simulink model "Thermal_Model_v5"  (R2026a)
settings: Solver=ode23t  StopTime=900
model workspace (MAT data in the model file):
  Area_coolant_bottom_port_in_m2 = 7.85398163397e-05
  Area_coolant_top_port_in_m2 = 7.85398163397e-05
  CurrentProfile = [0  80; 300  80; 300  0; 600  0; 600  -80; 900  -80]
  SOC0 = 0.4
  T_ambient_K = 298.15
  T_coolant_bottom_in_K = 298.15
  T_coolant_top_in_K = 298.15
  mdot_coolant_bottom = 0.02
  mdot_coolant_top = 0.02
libraries: fl_lib x24, nesl_utility x21, ThermalPackComponents_lib x6, batt_lib x6, SimscapeFluids_lib x6, Cylindrical_Cell_Module_v2_5_lib x1
settings Model: LastModifiedBy=Talha

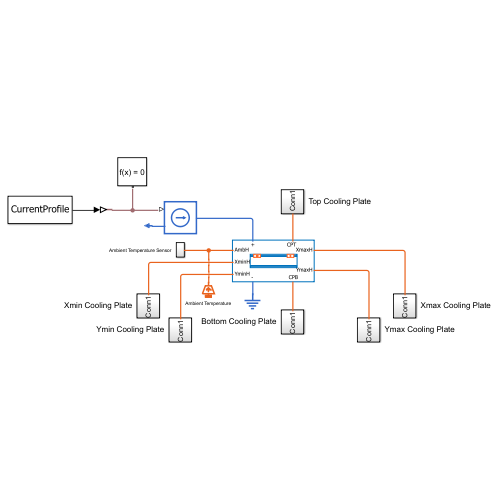
[thumbnail: Simulink's stored preview of the top-level diagram]
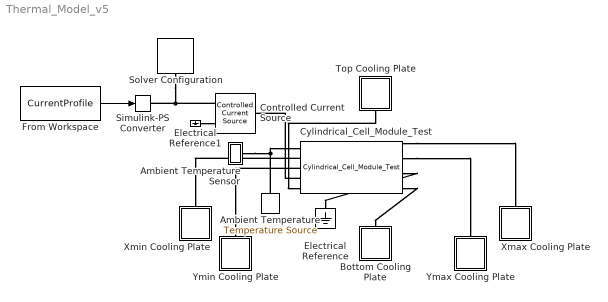
== system Thermal_Model_v5 ==
  Ambient Temperature : fl_lib/Thermal/Thermal Sources/Temperature Source  temperature=T_ambient_K K
  Ambient Temperature Sensor : Subsystem
  Bottom Cooling Plate : Subsystem
  Controlled Current Source : fl_lib/Electrical/Electrical Sources/Controlled Current Source
  Cylindrical_Cell_Module_Test : Cylindrical_Cell_Module_v2_5_lib/Cylindrical_Cell_Module_Test  BatteryCapacityCell=5 A*hr  BatteryCapacityCellPercentDeviation=zeros([12, 1])  ExtrapolationMethodCell=simscape.enum.extrapolation.nearest  SOCBreakpointsCell=[0, .1, .25, .5, .75, .9, 1]  SOCBreakpointsCellPercentDeviation=zeros([12, 1])  TemperatureBreakpointsCell=[278, 293, 313] K  TemperatureBreakpointsCellPercentDeviation=zeros([12, 1])  OpenCircuitVoltageThermalCell=[3.49, 3.5, 3.51; 3.55, 3.57, 3.56; 3.62, 3.63, 3.64; 3.71, 3.71, 3.72; 3.91, 3.93, 3.94; 4.07, 4.08, 4.08; 4.19, 4.19, 4.19] V  OpenCircuitVoltageThermalCellPercentDeviation=zeros([12, 1])  VoltageRangeCell=[0, inf] V  VoltageRangeCellPercentDeviation=zeros([12, 1])  ResistanceSOCBreakpointsCell=[0, .1, .25, .5, .75, .9, 1]  ResistanceSOCBreakpointsCellPercentDeviation=zeros([12, 1])  ResistanceTemperatureBreakpointsCell=[278, 293, 313] K  ResistanceTemperatureBreakpointsCellPercentDeviation=zeros([12, 1])  R0ThermalCell=[.0117, .0085, .009; .011, .0085, .009; .0114, .0087, .0092; .0107, .0082, .0088; .0107, .0083, .0091; .0113, .0085, .0089; .0116, .0085, .0089] Ohm  R0ThermalCellPercentDeviation=zeros([12, 1])  BatteryThermalMassCell=100 J/K  BatteryThermalMassCellPercentDeviation=zeros([12, 1])  NumThermalModelsCell=6  NumThermalModelsCellPercentDeviation=zeros([12, 1])  ThermalConductivityZCell=15 W/(K*m)  ThermalConductivityZCellPercentDeviation=zeros([12, 1])  CrossSectionalAreaXYCell=3.142e-4 m^2  CrossSectionalAreaXYCellPercentDeviation=zeros([12, 1])  HeightCell=0.07 m  HeightCellPercentDeviation=zeros([12, 1])  CoolantResistance=1.2 K/W  AmbientResistance=25 K/W  XminThermalResistance=25 K/W  XmaxThermalResistance=25 K/W  YminThermalResistance=25 K/W  YmaxThermalResistance=25 K/W  InterCellThermalResistance=1 K/W  InterParallelAssemblyThermalResistance=1 K/W  socCell_specify=on  socCell_priority=High  socCell=repmat(0.4, 12, 1)  socCell_nominal_specify=off  socCell_nominal_value=1  socCell_nominal_unit=1  batteryVoltage_specify=off  batteryVoltage_priority=None  batteryVoltage=repmat(0, 12, 1) V  batteryVoltage_nominal_specify=off  batteryVoltage_nominal_value=1  batteryVoltage_nominal_unit=V  batteryCurrent_specify=off  batteryCurrent_priority=None  batteryCurrent=repmat(0, 12, 1) A  batteryCurrent_nominal_specify=off  batteryCurrent_nominal_value=1  batteryCurrent_nominal_unit=A  numCycles_specify=off  numCycles_priority=High  numCycles=repmat(0, 12, 1)  numCycles_nominal_specify=off  numCycles_nominal_value=1  numCycles_nominal_unit=1  batteryTemperature_specify=on  batteryTemperature_priority=High  batteryTemperature=repmat(298.15, 12, 1) K  batteryTemperature_nominal_specify=off  batteryTemperature_nominal_value=1  batteryTemperature_nominal_unit=K  vParallelAssembly_specify=off  vParallelAssembly_priority=None  vParallelAssembly=repmat(0, 3, 1) V  vParallelAssembly_nominal_specify=off  vParallelAssembly_nominal_value=1  vParallelAssembly_nominal_unit=V  socParallelAssembly_specify=off  socParallelAssembly_priority=None  socParallelAssembly=repmat(1, 3, 1)  socParallelAssembly_nominal_specify=off  socParallelAssembly_nominal_value=1  socParallelAssembly_nominal_unit=1
  Electrical Reference : fl_lib/Electrical/Electrical Elements/Electrical Reference
  Electrical Reference1 : fl_lib/Electrical/Electrical Elements/Electrical Reference
  From Workspace : FromWorkspace  VariableName=CurrentProfile  Interpolate=off  OutputAfterFinalValue=Holding final value
  Simulink-PS Converter : nesl_utility/Simulink-PS Converter  PhysicalDomain=network_engine_domain  SubClassName=ps_input  LeftPortType=input  RightPortType=output  PseudoPeriodic=off  Frequencies=[]  NoiseDistribution=none  NoiseParameters=[]  Unit=1  AffineConversion=off  FilteringAndDerivatives=provide  SimscapeFilterOrder=1  InputFilterTimeConstant=0.001  UdotUserProvided=0
  Solver Configuration : nesl_utility/Solver Configuration  PhysicalDomain=network_engine_domain  SubClassName=solver  LeftPortType=input  RightPortType=generic  Tones=[]  Harmonics=[]  SimulateNoise=off  Profile=off  UseLocalSampling=off  EnableSwitchedLinearOptims=on  FrequencyDomain=off  UseCCode=off  RelTol=0.001  AbsTol=0.001  MinStep=1e-09  ToWorkspace=off  RevertToSquareIcSolve=off  NumHomotopyIterations=100  PhasorMode=off  PhasorModeNumHarmonics=1  ConsistencySolver=NEWTON_XTOL_AFTER_FTOL  CanonicalOrdering=CANONICAL  OptimizeIntermediates=OPTIMIZED  IndexReductionMethod=DerivativeReplacement  DoDC=off  ResidualTolerance=1e-09  ConsistencyTolSource=GLOBAL  ConsistencyAbsTol=0.001  ConsistencyRelTol=0.001  ConsistencyTolFactor=0.001  UseLocalSolver=off  LocalSolverChoice=NE_BACKWARD_EULER_ADVANCER  ResolveIndetEquations=on  FunctionEvalNumThread=1  LocalSolverSampleTime=0.001  DoFixedCost=off  MaxNonlinIter=3  MaxModeIter=2  ComputeImpulses=off  ImpulseIterations=2  LinearAlgebra=auto  LinearAlgebraNumThread=0  EquationFormulation=NE_TIME_EF  DelaysMemoryBudget=1024  AutomaticFiltering=on  FilteringTimeConstant=0.001  PartitionStorageMethod=AS_NEEDED  PartitionMemoryBudget=1024  PartitionMethod=ROBUST  MultibodyUseLocalSolver=off  MultibodyLocalSolverChoice=ODE1  MultibodyLocalSolverSampleTime=0.001
  Top Cooling Plate : Subsystem
  Xmax Cooling Plate : Subsystem
  Xmin Cooling Plate : Subsystem
  Ymax Cooling Plate : Subsystem
  Ymin Cooling Plate : Subsystem
  wires:
  From Workspace/1 -> Simulink-PS Converter/1
  connections:
  Controlled Current Source/RConn1 -- Solver Configuration/RConn1 -- Simulink-PS Converter/RConn1
  Cylindrical_Cell_Module_Test/RConn3 -- Electrical Reference/LConn1
  Cylindrical_Cell_Module_Test/LConn4 -- Controlled Current Source/LConn1
  Electrical Reference1/LConn1 -- Controlled Current Source/RConn2
  Ambient Temperature Sensor/LConn1 -- Ambient Temperature/LConn1 -- Cylindrical_Cell_Module_Test/LConn1
  Top Cooling Plate/LConn1 -- Cylindrical_Cell_Module_Test/LConn5
  Cylindrical_Cell_Module_Test/RConn4 -- Bottom Cooling Plate/LConn1
  Cylindrical_Cell_Module_Test/LConn2 -- Xmin Cooling Plate/LConn1
  Cylindrical_Cell_Module_Test/LConn3 -- Ymin Cooling Plate/LConn1
  Cylindrical_Cell_Module_Test/RConn1 -- Xmax Cooling Plate/LConn1
  Cylindrical_Cell_Module_Test/RConn2 -- Ymax Cooling Plate/LConn1

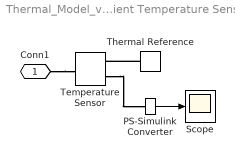
== system Thermal_Model_v5/Ambient Temperature Sensor ==
  PS-Simulink Converter : nesl_utility/PS-Simulink Converter  PhysicalDomain=network_engine_domain  SubClassName=ps_output  LeftPortType=input  RightPortType=output  PseudoPeriodic=off  Frequencies=[]  VectorFormat=inherit  Unit=inherit  AffineConversion=off
  Scope : Scope
      settings: ActiveDisplayYMinimum=-1  ActiveDisplayYMaximum=1
  Temperature Sensor : fl_lib/Thermal/Thermal Sensors/Temperature Sensor  temperature_measure=foundation.enum.MeasurementReference.difference
  Thermal Reference : fl_lib/Thermal/Thermal Elements/Thermal Reference
  Conn1 : PMIOPort  Side=Left
  wires:
  PS-Simulink Converter/1 -> Scope/1
  connections:
  Thermal Reference/LConn1 -- Temperature Sensor/RConn1
  Temperature Sensor/RConn2 -- PS-Simulink Converter/LConn1
  Conn1/RConn1 -- Temperature Sensor/LConn1

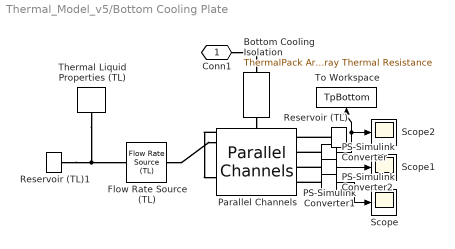
== system Thermal_Model_v5/Bottom Cooling Plate ==
  Bottom Cooling Isolation : ThermalPackComponents_lib/ThermalPack Array Thermal Resistance  N=12  R=1e-6 K/W
  Flow Rate Source (TL) : fl_lib/Thermal Liquid/Sources/Flow Rate Source (TL)  source_type=foundation.enum.constant_controlled.constant  flow_type=foundation.enum.mass_volumetric_flow.mass  mass_flow=mdot_coolant_bottom kg/s  volumetric_flow=0 m^3/s  power_spec=foundation.enum.power_spec.none  area=Area_coolant_bottom_port_in_m2 m^2
  PS-Simulink Converter : nesl_utility/PS-Simulink Converter  PhysicalDomain=network_engine_domain  SubClassName=ps_output  LeftPortType=input  RightPortType=output  PseudoPeriodic=off  Frequencies=[]  VectorFormat=inherit  Unit=inherit  AffineConversion=off
  PS-Simulink Converter1 : nesl_utility/PS-Simulink Converter  PhysicalDomain=network_engine_domain  SubClassName=ps_output  LeftPortType=input  RightPortType=output  PseudoPeriodic=off  Frequencies=[]  VectorFormat=inherit  Unit=inherit  AffineConversion=off
  PS-Simulink Converter2 : nesl_utility/PS-Simulink Converter  PhysicalDomain=network_engine_domain  SubClassName=ps_output  LeftPortType=input  RightPortType=output  PseudoPeriodic=off  Frequencies=[]  VectorFormat=inherit  Unit=inherit  AffineConversion=off
  Parallel Channels : batt_lib/Thermal/Parallel Channels  plateConnectivity=simscape.battery.enum.thermal.coolingPlateConnectivity.singleSided  numBattThermalNodes1=12  dimensionThermalNodes1=[0.0200 0.0200; 0.0200 0.0200; 0.0200 0.0200; 0.0200 0.0200; 0.0200 0.0200; 0.0200 0.0200; 0.0200 0.0200; 0.0200 0.0200; 0.0200 0.0200; 0.0200 0.0200; 0.0200 0.0200; 0.0200 0.0200]  locationThermalNodes1=[0.0100 0.0100; 0.0100 0.0310; 0.0100 0.0520; 0.0100 0.0730; 0.0310 0.0100; 0.0310 0.0310; 0.0310 0.0520; 0.0310 0.0730; 0.0520 0.0100; 0.0520 0.0310; 0.0520 0.0520; 0.0520 0.0730]  numBattThermalNodes2=1  dimensionThermalNodes2=ones(1, 2)  locationThermalNodes2=ones(1, 2)  plateDimX=3  plateDimY=4  plateTh=2e-3 m  plateThCond=205 W/(K*m)  plateDen=2700 kg/m^3  plateCp=900 J/(K*kg)  plateTemp_ini=298.15 K  Re_lam=2000  Re_tur=4000  Nu_lam=3.66  length_add=1e-3 m  shape_factor=64  nChannels=4  selectChannelOrientation=simscape.battery.enum.thermal.coolingChannelsDirection.alongX  channelDia=0.004 m  distributorDia=0.006 m  roughnessPipe=1.5e-05 m
  Reservoir (TL) : fl_lib/Thermal Liquid/Elements/Reservoir (TL)  pressure_input=false  pressure_spec=foundation.enum.pressure_spec.atmospheric  reservoir_pressure=101325 Pa  temperature_input=false  reservoir_temperature=298.15 K  area=Area_coolant_bottom_port_in_m2 m^2  input_error_spec=foundation.enum.input_range_error.warn
  Reservoir (TL)1 : fl_lib/Thermal Liquid/Elements/Reservoir (TL)  pressure_input=false  pressure_spec=foundation.enum.pressure_spec.atmospheric  reservoir_pressure=101325 Pa  temperature_input=false  reservoir_temperature=T_coolant_bottom_in_K K  area=Area_coolant_bottom_port_in_m2 m^2  input_error_spec=foundation.enum.input_range_error.warn
  Scope : Scope
      settings: ActiveDisplayYMinimum=-5455.2115602984395  ActiveDisplayYMaximum=-5434.2762079587283
  Scope1 : Scope
      settings: ActiveDisplayYMinimum=-1  ActiveDisplayYMaximum=1  DataLoggingVariableName=ScopeData2
  Scope2 : Scope
      settings: ActiveDisplayYMinimum=300.00863941911916  ActiveDisplayYMaximum=300.14142336544342  DataLoggingVariableName=ScopeData3
  Thermal Liquid Properties (TL) : SimscapeFluids_lib/Thermal Liquid/Utilities/Thermal Liquid Properties (TL)  fluid_list=fluids.thermal_liquid.utilities.enum.thermal_liquid_fluid_list.ethylene_glycol  concentration_param_EG=fluids.thermal_liquid.utilities.enum.thermal_liquid_concentration.volume_fraction  concentration_param_PG=fluids.thermal_liquid.utilities.enum.thermal_liquid_concentration.volume_fraction  c_mass_SW=3.5e-3  c_mass_EG=0.1  c_mass_PG=0.1  c_mass_GL=0.1  c_vol_EG=0.5  c_vol_PG=0.1  beta_const_EG=2.1791 GPa  beta_const_PG=2.1791 GPa  beta_const_GL=2.1791 GPa  p_min_EG=0.01 MPa  p_min_PG=0.01 MPa  p_min_GL=0.01 MPa  p_max_EG=50 MPa  p_max_PG=50 MPa  p_max_GL=50 MPa  T_atm=298.15 K  p_atm=0.101325 MPa  properties_range_check=simscape.enum.assert.action.error  air_fraction=0.005  R_air=0.287 kJ/(K*kg)  air_dissolution_model=false  p_crit=3 MPa
  To Workspace : ToWorkspace  VariableName=TpBottom  SaveFormat=Timeseries  SampleTime=-1
  Conn1 : PMIOPort  Side=Left
  wires:
  PS-Simulink Converter/1 -> Scope2/1, To Workspace/1
  PS-Simulink Converter1/1 -> Scope1/1
  PS-Simulink Converter2/1 -> Scope/1
  connections:
  PS-Simulink Converter2/LConn1 -- Parallel Channels/RConn4
  Reservoir (TL)1/LConn1 -- Thermal Liquid Properties (TL)/RConn1 -- Flow Rate Source (TL)/LConn1
  PS-Simulink Converter1/LConn1 -- Parallel Channels/RConn3
  PS-Simulink Converter/LConn1 -- Parallel Channels/RConn2
  Reservoir (TL)/LConn1 -- Parallel Channels/RConn1
  Bottom Cooling Isolation/RConn1 -- Parallel Channels/LConn2
  Flow Rate Source (TL)/RConn1 -- Parallel Channels/LConn1
  Conn1/RConn1 -- Bottom Cooling Isolation/LConn1

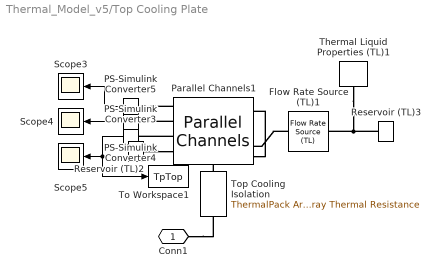
== system Thermal_Model_v5/Top Cooling Plate ==
  Flow Rate Source (TL)1 : fl_lib/Thermal Liquid/Sources/Flow Rate Source (TL)  source_type=foundation.enum.constant_controlled.constant  flow_type=foundation.enum.mass_volumetric_flow.mass  mass_flow=mdot_coolant_top kg/s  volumetric_flow=0 m^3/s  power_spec=foundation.enum.power_spec.none  area=Area_coolant_top_port_in_m2 m^2
  PS-Simulink Converter3 : nesl_utility/PS-Simulink Converter  PhysicalDomain=network_engine_domain  SubClassName=ps_output  LeftPortType=input  RightPortType=output  PseudoPeriodic=off  Frequencies=[]  VectorFormat=inherit  Unit=inherit  AffineConversion=off
  PS-Simulink Converter4 : nesl_utility/PS-Simulink Converter  PhysicalDomain=network_engine_domain  SubClassName=ps_output  LeftPortType=input  RightPortType=output  PseudoPeriodic=off  Frequencies=[]  VectorFormat=inherit  Unit=inherit  AffineConversion=off
  PS-Simulink Converter5 : nesl_utility/PS-Simulink Converter  PhysicalDomain=network_engine_domain  SubClassName=ps_output  LeftPortType=input  RightPortType=output  PseudoPeriodic=off  Frequencies=[]  VectorFormat=inherit  Unit=inherit  AffineConversion=off
  Parallel Channels1 : batt_lib/Thermal/Parallel Channels  plateConnectivity=simscape.battery.enum.thermal.coolingPlateConnectivity.singleSided  numBattThermalNodes1=12  dimensionThermalNodes1=[0.0200 0.0200; 0.0200 0.0200; 0.0200 0.0200; 0.0200 0.0200; 0.0200 0.0200; 0.0200 0.0200; 0.0200 0.0200; 0.0200 0.0200; 0.0200 0.0200; 0.0200 0.0200; 0.0200 0.0200; 0.0200 0.0200]  locationThermalNodes1=[0.0100 0.0100; 0.0100 0.0310; 0.0100 0.0520; 0.0100 0.0730; 0.0310 0.0100; 0.0310 0.0310; 0.0310 0.0520; 0.0310 0.0730; 0.0520 0.0100; 0.0520 0.0310; 0.0520 0.0520; 0.0520 0.0730]  numBattThermalNodes2=1  dimensionThermalNodes2=ones(1, 2)  locationThermalNodes2=ones(1, 2)  plateDimX=3  plateDimY=4  plateTh=2e-3 m  plateThCond=205 W/(K*m)  plateDen=2700 kg/m^3  plateCp=900 J/(K*kg)  plateTemp_ini=298.15 K  Re_lam=2000  Re_tur=4000  Nu_lam=3.66  length_add=1e-3 m  shape_factor=64  nChannels=4  selectChannelOrientation=simscape.battery.enum.thermal.coolingChannelsDirection.alongX  channelDia=0.004 m  distributorDia=0.006 m  roughnessPipe=1.5e-05 m
  Reservoir (TL)2 : fl_lib/Thermal Liquid/Elements/Reservoir (TL)  pressure_input=false  pressure_spec=foundation.enum.pressure_spec.atmospheric  reservoir_pressure=101325 Pa  temperature_input=false  reservoir_temperature=298.15 K  area=Area_coolant_top_port_in_m2 m^2  input_error_spec=foundation.enum.input_range_error.warn
  Reservoir (TL)3 : fl_lib/Thermal Liquid/Elements/Reservoir (TL)  pressure_input=false  pressure_spec=foundation.enum.pressure_spec.atmospheric  reservoir_pressure=101325 Pa  temperature_input=false  reservoir_temperature=T_coolant_top_in_K K  area=Area_coolant_top_port_in_m2 m^2  input_error_spec=foundation.enum.input_range_error.warn
  Scope3 : Scope
      settings: ActiveDisplayYMinimum=-5455.2115602984395  ActiveDisplayYMaximum=-5434.2762079587283  DataLoggingVariableName=ScopeData4
  Scope4 : Scope
      settings: ActiveDisplayYMinimum=-1  ActiveDisplayYMaximum=1  DataLoggingVariableName=ScopeData5
  Scope5 : Scope
      settings: ActiveDisplayYMinimum=300.00863941911916  ActiveDisplayYMaximum=300.14142336544342  DataLoggingVariableName=ScopeData6
  Thermal Liquid Properties (TL)1 : SimscapeFluids_lib/Thermal Liquid/Utilities/Thermal Liquid Properties (TL)  fluid_list=fluids.thermal_liquid.utilities.enum.thermal_liquid_fluid_list.ethylene_glycol  concentration_param_EG=fluids.thermal_liquid.utilities.enum.thermal_liquid_concentration.volume_fraction  concentration_param_PG=fluids.thermal_liquid.utilities.enum.thermal_liquid_concentration.volume_fraction  c_mass_SW=3.5e-3  c_mass_EG=0.1  c_mass_PG=0.1  c_mass_GL=0.1  c_vol_EG=0.5  c_vol_PG=0.1  beta_const_EG=2.1791 GPa  beta_const_PG=2.1791 GPa  beta_const_GL=2.1791 GPa  p_min_EG=0.01 MPa  p_min_PG=0.01 MPa  p_min_GL=0.01 MPa  p_max_EG=50 MPa  p_max_PG=50 MPa  p_max_GL=50 MPa  T_atm=298.15 K  p_atm=0.101325 MPa  properties_range_check=simscape.enum.assert.action.error  air_fraction=0.005  R_air=0.287 kJ/(K*kg)  air_dissolution_model=false  p_crit=3 MPa
  To Workspace1 : ToWorkspace  VariableName=TpTop  SaveFormat=Timeseries  SampleTime=-1
  Top Cooling Isolation : ThermalPackComponents_lib/ThermalPack Array Thermal Resistance  N=12  R=1e9 K/W
  Conn1 : PMIOPort  Side=Left
  wires:
  PS-Simulink Converter3/1 -> To Workspace1/1, Scope5/1
  PS-Simulink Converter5/1 -> Scope3/1
  PS-Simulink Converter4/1 -> Scope4/1
  connections:
  Reservoir (TL)2/LConn1 -- Parallel Channels1/RConn1
  Parallel Channels1/RConn4 -- PS-Simulink Converter5/LConn1
  Thermal Liquid Properties (TL)1/RConn1 -- Reservoir (TL)3/LConn1 -- Flow Rate Source (TL)1/LConn1
  Parallel Channels1/RConn3 -- PS-Simulink Converter4/LConn1
  Top Cooling Isolation/RConn1 -- Parallel Channels1/LConn2
  Parallel Channels1/RConn2 -- PS-Simulink Converter3/LConn1
  Flow Rate Source (TL)1/RConn1 -- Parallel Channels1/LConn1
  Conn1/RConn1 -- Top Cooling Isolation/LConn1

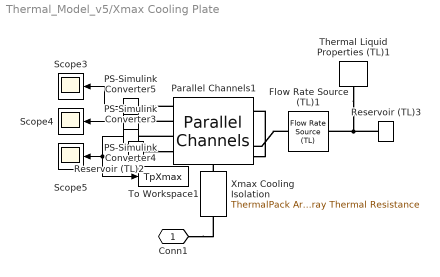
== system Thermal_Model_v5/Xmax Cooling Plate ==
  Flow Rate Source (TL)1 : fl_lib/Thermal Liquid/Sources/Flow Rate Source (TL)  source_type=foundation.enum.constant_controlled.constant  flow_type=foundation.enum.mass_volumetric_flow.mass  mass_flow=mdot_coolant_Xmax kg/s  volumetric_flow=0 m^3/s  power_spec=foundation.enum.power_spec.none  area=Area_coolant_Xmax_port_in_m2 m^2
  PS-Simulink Converter3 : nesl_utility/PS-Simulink Converter  PhysicalDomain=network_engine_domain  SubClassName=ps_output  LeftPortType=input  RightPortType=output  PseudoPeriodic=off  Frequencies=[]  VectorFormat=inherit  Unit=inherit  AffineConversion=off
  PS-Simulink Converter4 : nesl_utility/PS-Simulink Converter  PhysicalDomain=network_engine_domain  SubClassName=ps_output  LeftPortType=input  RightPortType=output  PseudoPeriodic=off  Frequencies=[]  VectorFormat=inherit  Unit=inherit  AffineConversion=off
  PS-Simulink Converter5 : nesl_utility/PS-Simulink Converter  PhysicalDomain=network_engine_domain  SubClassName=ps_output  LeftPortType=input  RightPortType=output  PseudoPeriodic=off  Frequencies=[]  VectorFormat=inherit  Unit=inherit  AffineConversion=off
  Parallel Channels1 : batt_lib/Thermal/Parallel Channels  plateConnectivity=simscape.battery.enum.thermal.coolingPlateConnectivity.singleSided  numBattThermalNodes1=4  dimensionThermalNodes1=|  locationThermalNodes1=|  numBattThermalNodes2=1  dimensionThermalNodes2=ones(1, 2)  locationThermalNodes2=ones(1, 2)  plateDimX=3  plateDimY=4  plateTh=2e-3 m  plateThCond=205 W/(K*m)  plateDen=2700 kg/m^3  plateCp=900 J/(K*kg)  plateTemp_ini=298.15 K  Re_lam=2000  Re_tur=4000  Nu_lam=3.66  length_add=1e-3 m  shape_factor=64  nChannels=4  selectChannelOrientation=simscape.battery.enum.thermal.coolingChannelsDirection.alongX  channelDia=0.004 m  distributorDia=0.006 m  roughnessPipe=1.5e-05 m
      dimensionThermalNodes1=|
      | [0.0700 0.0314; 0.0700 0.0314; 0.0700 0.0314;
      | 0.0700 0.0314]
      locationThermalNodes1=|
      | [0.0350 0.0100;
      | 0.0350 0.0310;
      | 0.0350 0.0520;
      | 0.0350 0.0730]
  Reservoir (TL)2 : fl_lib/Thermal Liquid/Elements/Reservoir (TL)  pressure_input=false  pressure_spec=foundation.enum.pressure_spec.atmospheric  reservoir_pressure=101325 Pa  temperature_input=false  reservoir_temperature=298.15 K  area=Area_coolant_Xmax_port_in_m2 m^2  input_error_spec=foundation.enum.input_range_error.warn
  Reservoir (TL)3 : fl_lib/Thermal Liquid/Elements/Reservoir (TL)  pressure_input=false  pressure_spec=foundation.enum.pressure_spec.atmospheric  reservoir_pressure=101325 Pa  temperature_input=false  reservoir_temperature=T_coolant_Xmax_in_K K  area=Area_coolant_Xmax_port_in_m2 m^2  input_error_spec=foundation.enum.input_range_error.warn
  Scope3 : Scope
      settings: ActiveDisplayYMinimum=-5455.2115602984395  ActiveDisplayYMaximum=-5434.2762079587283  DataLoggingVariableName=ScopeData4
  Scope4 : Scope
      settings: ActiveDisplayYMinimum=-1  ActiveDisplayYMaximum=1  DataLoggingVariableName=ScopeData5
  Scope5 : Scope
      settings: ActiveDisplayYMinimum=300.00863941911916  ActiveDisplayYMaximum=300.14142336544342  DataLoggingVariableName=ScopeData6
  Thermal Liquid Properties (TL)1 : SimscapeFluids_lib/Thermal Liquid/Utilities/Thermal Liquid Properties (TL)  fluid_list=fluids.thermal_liquid.utilities.enum.thermal_liquid_fluid_list.ethylene_glycol  concentration_param_EG=fluids.thermal_liquid.utilities.enum.thermal_liquid_concentration.volume_fraction  concentration_param_PG=fluids.thermal_liquid.utilities.enum.thermal_liquid_concentration.volume_fraction  c_mass_SW=3.5e-3  c_mass_EG=0.1  c_mass_PG=0.1  c_mass_GL=0.1  c_vol_EG=0.5  c_vol_PG=0.1  beta_const_EG=2.1791 GPa  beta_const_PG=2.1791 GPa  beta_const_GL=2.1791 GPa  p_min_EG=0.01 MPa  p_min_PG=0.01 MPa  p_min_GL=0.01 MPa  p_max_EG=50 MPa  p_max_PG=50 MPa  p_max_GL=50 MPa  T_atm=298.15 K  p_atm=0.101325 MPa  properties_range_check=simscape.enum.assert.action.error  air_fraction=0.005  R_air=0.287 kJ/(K*kg)  air_dissolution_model=false  p_crit=3 MPa
  To Workspace1 : ToWorkspace  VariableName=TpXmax  SaveFormat=Timeseries  SampleTime=-1
  Xmax Cooling Isolation : ThermalPackComponents_lib/ThermalPack Array Thermal Resistance  N=4  R=1e9 K/W
  Conn1 : PMIOPort  Side=Left
  wires:
  PS-Simulink Converter3/1 -> To Workspace1/1, Scope5/1
  PS-Simulink Converter5/1 -> Scope3/1
  PS-Simulink Converter4/1 -> Scope4/1
  connections:
  Reservoir (TL)2/LConn1 -- Parallel Channels1/RConn1
  Parallel Channels1/RConn4 -- PS-Simulink Converter5/LConn1
  Thermal Liquid Properties (TL)1/RConn1 -- Reservoir (TL)3/LConn1 -- Flow Rate Source (TL)1/LConn1
  Parallel Channels1/RConn3 -- PS-Simulink Converter4/LConn1
  Xmax Cooling Isolation/RConn1 -- Parallel Channels1/LConn2
  Parallel Channels1/RConn2 -- PS-Simulink Converter3/LConn1
  Flow Rate Source (TL)1/RConn1 -- Parallel Channels1/LConn1
  Conn1/RConn1 -- Xmax Cooling Isolation/LConn1

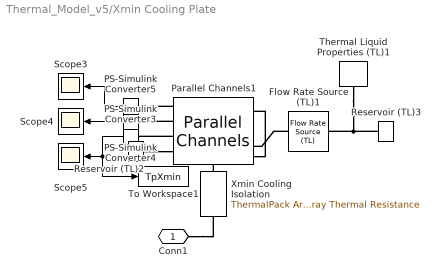
== system Thermal_Model_v5/Xmin Cooling Plate ==
  Flow Rate Source (TL)1 : fl_lib/Thermal Liquid/Sources/Flow Rate Source (TL)  source_type=foundation.enum.constant_controlled.constant  flow_type=foundation.enum.mass_volumetric_flow.mass  mass_flow=mdot_coolant_Xmin kg/s  volumetric_flow=0 m^3/s  power_spec=foundation.enum.power_spec.none  area=Area_coolant_Xmin_port_in_m2 m^2
  PS-Simulink Converter3 : nesl_utility/PS-Simulink Converter  PhysicalDomain=network_engine_domain  SubClassName=ps_output  LeftPortType=input  RightPortType=output  PseudoPeriodic=off  Frequencies=[]  VectorFormat=inherit  Unit=inherit  AffineConversion=off
  PS-Simulink Converter4 : nesl_utility/PS-Simulink Converter  PhysicalDomain=network_engine_domain  SubClassName=ps_output  LeftPortType=input  RightPortType=output  PseudoPeriodic=off  Frequencies=[]  VectorFormat=inherit  Unit=inherit  AffineConversion=off
  PS-Simulink Converter5 : nesl_utility/PS-Simulink Converter  PhysicalDomain=network_engine_domain  SubClassName=ps_output  LeftPortType=input  RightPortType=output  PseudoPeriodic=off  Frequencies=[]  VectorFormat=inherit  Unit=inherit  AffineConversion=off
  Parallel Channels1 : batt_lib/Thermal/Parallel Channels  plateConnectivity=simscape.battery.enum.thermal.coolingPlateConnectivity.singleSided  numBattThermalNodes1=4  dimensionThermalNodes1=|  locationThermalNodes1=|  numBattThermalNodes2=1  dimensionThermalNodes2=ones(1, 2)  locationThermalNodes2=ones(1, 2)  plateDimX=3  plateDimY=4  plateTh=2e-3 m  plateThCond=205 W/(K*m)  plateDen=2700 kg/m^3  plateCp=900 J/(K*kg)  plateTemp_ini=298.15 K  Re_lam=2000  Re_tur=4000  Nu_lam=3.66  length_add=1e-3 m  shape_factor=64  nChannels=4  selectChannelOrientation=simscape.battery.enum.thermal.coolingChannelsDirection.alongX  channelDia=0.004 m  distributorDia=0.006 m  roughnessPipe=1.5e-05 m
      dimensionThermalNodes1=|
      | [0.0700 0.0314; 0.0700 0.0314; 0.0700 0.0314;
      | 0.0700 0.0314]
      locationThermalNodes1=|
      | [0.0350 0.0100;
      | 0.0350 0.0310;
      | 0.0350 0.0520;
      | 0.0350 0.0730]
  Reservoir (TL)2 : fl_lib/Thermal Liquid/Elements/Reservoir (TL)  pressure_input=false  pressure_spec=foundation.enum.pressure_spec.atmospheric  reservoir_pressure=101325 Pa  temperature_input=false  reservoir_temperature=298.15 K  area=Area_coolant_Xmin_port_in_m2 m^2  input_error_spec=foundation.enum.input_range_error.warn
  Reservoir (TL)3 : fl_lib/Thermal Liquid/Elements/Reservoir (TL)  pressure_input=false  pressure_spec=foundation.enum.pressure_spec.atmospheric  reservoir_pressure=101325 Pa  temperature_input=false  reservoir_temperature=T_coolant_Xmin_in_K K  area=Area_coolant_Xmin_port_in_m2 m^2  input_error_spec=foundation.enum.input_range_error.warn
  Scope3 : Scope
      settings: ActiveDisplayYMinimum=-5455.2115602984395  ActiveDisplayYMaximum=-5434.2762079587283  DataLoggingVariableName=ScopeData4
  Scope4 : Scope
      settings: ActiveDisplayYMinimum=-1  ActiveDisplayYMaximum=1  DataLoggingVariableName=ScopeData5
  Scope5 : Scope
      settings: ActiveDisplayYMinimum=300.00863941911916  ActiveDisplayYMaximum=300.14142336544342  DataLoggingVariableName=ScopeData6
  Thermal Liquid Properties (TL)1 : SimscapeFluids_lib/Thermal Liquid/Utilities/Thermal Liquid Properties (TL)  fluid_list=fluids.thermal_liquid.utilities.enum.thermal_liquid_fluid_list.ethylene_glycol  concentration_param_EG=fluids.thermal_liquid.utilities.enum.thermal_liquid_concentration.volume_fraction  concentration_param_PG=fluids.thermal_liquid.utilities.enum.thermal_liquid_concentration.volume_fraction  c_mass_SW=3.5e-3  c_mass_EG=0.1  c_mass_PG=0.1  c_mass_GL=0.1  c_vol_EG=0.5  c_vol_PG=0.1  beta_const_EG=2.1791 GPa  beta_const_PG=2.1791 GPa  beta_const_GL=2.1791 GPa  p_min_EG=0.01 MPa  p_min_PG=0.01 MPa  p_min_GL=0.01 MPa  p_max_EG=50 MPa  p_max_PG=50 MPa  p_max_GL=50 MPa  T_atm=298.15 K  p_atm=0.101325 MPa  properties_range_check=simscape.enum.assert.action.error  air_fraction=0.005  R_air=0.287 kJ/(K*kg)  air_dissolution_model=false  p_crit=3 MPa
  To Workspace1 : ToWorkspace  VariableName=TpXmin  SaveFormat=Timeseries  SampleTime=-1
  Xmin Cooling Isolation : ThermalPackComponents_lib/ThermalPack Array Thermal Resistance  N=4  R=1e9 K/W
  Conn1 : PMIOPort  Side=Left
  wires:
  PS-Simulink Converter3/1 -> To Workspace1/1, Scope5/1
  PS-Simulink Converter5/1 -> Scope3/1
  PS-Simulink Converter4/1 -> Scope4/1
  connections:
  Reservoir (TL)2/LConn1 -- Parallel Channels1/RConn1
  Parallel Channels1/RConn4 -- PS-Simulink Converter5/LConn1
  Thermal Liquid Properties (TL)1/RConn1 -- Reservoir (TL)3/LConn1 -- Flow Rate Source (TL)1/LConn1
  Parallel Channels1/RConn3 -- PS-Simulink Converter4/LConn1
  Xmin Cooling Isolation/RConn1 -- Parallel Channels1/LConn2
  Parallel Channels1/RConn2 -- PS-Simulink Converter3/LConn1
  Flow Rate Source (TL)1/RConn1 -- Parallel Channels1/LConn1
  Conn1/RConn1 -- Xmin Cooling Isolation/LConn1

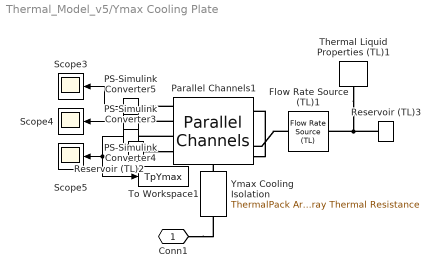
== system Thermal_Model_v5/Ymax Cooling Plate ==
  Flow Rate Source (TL)1 : fl_lib/Thermal Liquid/Sources/Flow Rate Source (TL)  source_type=foundation.enum.constant_controlled.constant  flow_type=foundation.enum.mass_volumetric_flow.mass  mass_flow=mdot_coolant_Ymax kg/s  volumetric_flow=0 m^3/s  power_spec=foundation.enum.power_spec.none  area=Area_coolant_Ymax_port_in_m2 m^2
  PS-Simulink Converter3 : nesl_utility/PS-Simulink Converter  PhysicalDomain=network_engine_domain  SubClassName=ps_output  LeftPortType=input  RightPortType=output  PseudoPeriodic=off  Frequencies=[]  VectorFormat=inherit  Unit=inherit  AffineConversion=off
  PS-Simulink Converter4 : nesl_utility/PS-Simulink Converter  PhysicalDomain=network_engine_domain  SubClassName=ps_output  LeftPortType=input  RightPortType=output  PseudoPeriodic=off  Frequencies=[]  VectorFormat=inherit  Unit=inherit  AffineConversion=off
  PS-Simulink Converter5 : nesl_utility/PS-Simulink Converter  PhysicalDomain=network_engine_domain  SubClassName=ps_output  LeftPortType=input  RightPortType=output  PseudoPeriodic=off  Frequencies=[]  VectorFormat=inherit  Unit=inherit  AffineConversion=off
  Parallel Channels1 : batt_lib/Thermal/Parallel Channels  plateConnectivity=simscape.battery.enum.thermal.coolingPlateConnectivity.singleSided  numBattThermalNodes1=3  dimensionThermalNodes1=|  locationThermalNodes1=|  numBattThermalNodes2=1  dimensionThermalNodes2=ones(1, 2)  locationThermalNodes2=ones(1, 2)  plateDimX=3  plateDimY=4  plateTh=2e-3 m  plateThCond=205 W/(K*m)  plateDen=2700 kg/m^3  plateCp=900 J/(K*kg)  plateTemp_ini=298.15 K  Re_lam=2000  Re_tur=4000  Nu_lam=3.66  length_add=1e-3 m  shape_factor=64  nChannels=4  selectChannelOrientation=simscape.battery.enum.thermal.coolingChannelsDirection.alongX  channelDia=0.004 m  distributorDia=0.006 m  roughnessPipe=1.5e-05 m
      dimensionThermalNodes1=|
      | [0.0700 0.0314;
      | 0.0700 0.0314; 0.0700 0.0314]
      locationThermalNodes1=|
      | [0.0350 0.0100; 0.0350 0.0310;
      | 0.0350 0.0520]
  Reservoir (TL)2 : fl_lib/Thermal Liquid/Elements/Reservoir (TL)  pressure_input=false  pressure_spec=foundation.enum.pressure_spec.atmospheric  reservoir_pressure=101325 Pa  temperature_input=false  reservoir_temperature=298.15 K  area=Area_coolant_Ymax_port_in_m2 m^2  input_error_spec=foundation.enum.input_range_error.warn
  Reservoir (TL)3 : fl_lib/Thermal Liquid/Elements/Reservoir (TL)  pressure_input=false  pressure_spec=foundation.enum.pressure_spec.atmospheric  reservoir_pressure=101325 Pa  temperature_input=false  reservoir_temperature=T_coolant_Ymax_in_K K  area=Area_coolant_Ymax_port_in_m2 m^2  input_error_spec=foundation.enum.input_range_error.warn
  Scope3 : Scope
      settings: ActiveDisplayYMinimum=-5455.2115602984395  ActiveDisplayYMaximum=-5434.2762079587283  DataLoggingVariableName=ScopeData4
  Scope4 : Scope
      settings: ActiveDisplayYMinimum=-1  ActiveDisplayYMaximum=1  DataLoggingVariableName=ScopeData5
  Scope5 : Scope
      settings: ActiveDisplayYMinimum=300.00863941911916  ActiveDisplayYMaximum=300.14142336544342  DataLoggingVariableName=ScopeData6
  Thermal Liquid Properties (TL)1 : SimscapeFluids_lib/Thermal Liquid/Utilities/Thermal Liquid Properties (TL)  fluid_list=fluids.thermal_liquid.utilities.enum.thermal_liquid_fluid_list.ethylene_glycol  concentration_param_EG=fluids.thermal_liquid.utilities.enum.thermal_liquid_concentration.volume_fraction  concentration_param_PG=fluids.thermal_liquid.utilities.enum.thermal_liquid_concentration.volume_fraction  c_mass_SW=3.5e-3  c_mass_EG=0.1  c_mass_PG=0.1  c_mass_GL=0.1  c_vol_EG=0.5  c_vol_PG=0.1  beta_const_EG=2.1791 GPa  beta_const_PG=2.1791 GPa  beta_const_GL=2.1791 GPa  p_min_EG=0.01 MPa  p_min_PG=0.01 MPa  p_min_GL=0.01 MPa  p_max_EG=50 MPa  p_max_PG=50 MPa  p_max_GL=50 MPa  T_atm=298.15 K  p_atm=0.101325 MPa  properties_range_check=simscape.enum.assert.action.error  air_fraction=0.005  R_air=0.287 kJ/(K*kg)  air_dissolution_model=false  p_crit=3 MPa
  To Workspace1 : ToWorkspace  VariableName=TpYmax  SaveFormat=Timeseries  SampleTime=-1
  Ymax Cooling Isolation : ThermalPackComponents_lib/ThermalPack Array Thermal Resistance  N=3  R=1e9 K/W
  Conn1 : PMIOPort  Side=Left
  wires:
  PS-Simulink Converter3/1 -> To Workspace1/1, Scope5/1
  PS-Simulink Converter5/1 -> Scope3/1
  PS-Simulink Converter4/1 -> Scope4/1
  connections:
  Reservoir (TL)2/LConn1 -- Parallel Channels1/RConn1
  Parallel Channels1/RConn4 -- PS-Simulink Converter5/LConn1
  Thermal Liquid Properties (TL)1/RConn1 -- Reservoir (TL)3/LConn1 -- Flow Rate Source (TL)1/LConn1
  Parallel Channels1/RConn3 -- PS-Simulink Converter4/LConn1
  Ymax Cooling Isolation/RConn1 -- Parallel Channels1/LConn2
  Parallel Channels1/RConn2 -- PS-Simulink Converter3/LConn1
  Flow Rate Source (TL)1/RConn1 -- Parallel Channels1/LConn1
  Conn1/RConn1 -- Ymax Cooling Isolation/LConn1

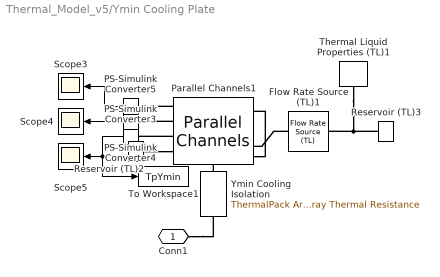
== system Thermal_Model_v5/Ymin Cooling Plate ==
  Flow Rate Source (TL)1 : fl_lib/Thermal Liquid/Sources/Flow Rate Source (TL)  source_type=foundation.enum.constant_controlled.constant  flow_type=foundation.enum.mass_volumetric_flow.mass  mass_flow=mdot_coolant_Ymin kg/s  volumetric_flow=0 m^3/s  power_spec=foundation.enum.power_spec.none  area=Area_coolant_Ymin_port_in_m2 m^2
  PS-Simulink Converter3 : nesl_utility/PS-Simulink Converter  PhysicalDomain=network_engine_domain  SubClassName=ps_output  LeftPortType=input  RightPortType=output  PseudoPeriodic=off  Frequencies=[]  VectorFormat=inherit  Unit=inherit  AffineConversion=off
  PS-Simulink Converter4 : nesl_utility/PS-Simulink Converter  PhysicalDomain=network_engine_domain  SubClassName=ps_output  LeftPortType=input  RightPortType=output  PseudoPeriodic=off  Frequencies=[]  VectorFormat=inherit  Unit=inherit  AffineConversion=off
  PS-Simulink Converter5 : nesl_utility/PS-Simulink Converter  PhysicalDomain=network_engine_domain  SubClassName=ps_output  LeftPortType=input  RightPortType=output  PseudoPeriodic=off  Frequencies=[]  VectorFormat=inherit  Unit=inherit  AffineConversion=off
  Parallel Channels1 : batt_lib/Thermal/Parallel Channels  plateConnectivity=simscape.battery.enum.thermal.coolingPlateConnectivity.singleSided  numBattThermalNodes1=3  dimensionThermalNodes1=|  locationThermalNodes1=|  numBattThermalNodes2=1  dimensionThermalNodes2=ones(1, 2)  locationThermalNodes2=ones(1, 2)  plateDimX=3  plateDimY=4  plateTh=2e-3 m  plateThCond=205 W/(K*m)  plateDen=2700 kg/m^3  plateCp=900 J/(K*kg)  plateTemp_ini=298.15 K  Re_lam=2000  Re_tur=4000  Nu_lam=3.66  length_add=1e-3 m  shape_factor=64  nChannels=4  selectChannelOrientation=simscape.battery.enum.thermal.coolingChannelsDirection.alongX  channelDia=0.004 m  distributorDia=0.006 m  roughnessPipe=1.5e-05 m
      dimensionThermalNodes1=|
      | [0.0700 0.0314;
      | 0.0700 0.0314; 0.0700 0.0314]
      locationThermalNodes1=|
      | [0.0350 0.0100; 0.0350 0.0310;
      | 0.0350 0.0520]
  Reservoir (TL)2 : fl_lib/Thermal Liquid/Elements/Reservoir (TL)  pressure_input=false  pressure_spec=foundation.enum.pressure_spec.atmospheric  reservoir_pressure=101325 Pa  temperature_input=false  reservoir_temperature=298.15 K  area=Area_coolant_Ymin_port_in_m2 m^2  input_error_spec=foundation.enum.input_range_error.warn
  Reservoir (TL)3 : fl_lib/Thermal Liquid/Elements/Reservoir (TL)  pressure_input=false  pressure_spec=foundation.enum.pressure_spec.atmospheric  reservoir_pressure=101325 Pa  temperature_input=false  reservoir_temperature=T_coolant_Ymin_in_K K  area=Area_coolant_Ymin_port_in_m2 m^2  input_error_spec=foundation.enum.input_range_error.warn
  Scope3 : Scope
      settings: ActiveDisplayYMinimum=-5455.2115602984395  ActiveDisplayYMaximum=-5434.2762079587283  DataLoggingVariableName=ScopeData4
  Scope4 : Scope
      settings: ActiveDisplayYMinimum=-1  ActiveDisplayYMaximum=1  DataLoggingVariableName=ScopeData5
  Scope5 : Scope
      settings: ActiveDisplayYMinimum=300.00863941911916  ActiveDisplayYMaximum=300.14142336544342  DataLoggingVariableName=ScopeData6
  Thermal Liquid Properties (TL)1 : SimscapeFluids_lib/Thermal Liquid/Utilities/Thermal Liquid Properties (TL)  fluid_list=fluids.thermal_liquid.utilities.enum.thermal_liquid_fluid_list.ethylene_glycol  concentration_param_EG=fluids.thermal_liquid.utilities.enum.thermal_liquid_concentration.volume_fraction  concentration_param_PG=fluids.thermal_liquid.utilities.enum.thermal_liquid_concentration.volume_fraction  c_mass_SW=3.5e-3  c_mass_EG=0.1  c_mass_PG=0.1  c_mass_GL=0.1  c_vol_EG=0.5  c_vol_PG=0.1  beta_const_EG=2.1791 GPa  beta_const_PG=2.1791 GPa  beta_const_GL=2.1791 GPa  p_min_EG=0.01 MPa  p_min_PG=0.01 MPa  p_min_GL=0.01 MPa  p_max_EG=50 MPa  p_max_PG=50 MPa  p_max_GL=50 MPa  T_atm=298.15 K  p_atm=0.101325 MPa  properties_range_check=simscape.enum.assert.action.error  air_fraction=0.005  R_air=0.287 kJ/(K*kg)  air_dissolution_model=false  p_crit=3 MPa
  To Workspace1 : ToWorkspace  VariableName=TpYmin  SaveFormat=Timeseries  SampleTime=-1
  Ymin Cooling Isolation : ThermalPackComponents_lib/ThermalPack Array Thermal Resistance  N=3  R=1e9 K/W
  Conn1 : PMIOPort  Side=Left
  wires:
  PS-Simulink Converter3/1 -> To Workspace1/1, Scope5/1
  PS-Simulink Converter5/1 -> Scope3/1
  PS-Simulink Converter4/1 -> Scope4/1
  connections:
  Reservoir (TL)2/LConn1 -- Parallel Channels1/RConn1
  Parallel Channels1/RConn4 -- PS-Simulink Converter5/LConn1
  Thermal Liquid Properties (TL)1/RConn1 -- Reservoir (TL)3/LConn1 -- Flow Rate Source (TL)1/LConn1
  Parallel Channels1/RConn3 -- PS-Simulink Converter4/LConn1
  Ymin Cooling Isolation/RConn1 -- Parallel Channels1/LConn2
  Parallel Channels1/RConn2 -- PS-Simulink Converter3/LConn1
  Flow Rate Source (TL)1/RConn1 -- Parallel Channels1/LConn1
  Conn1/RConn1 -- Ymin Cooling Isolation/LConn1
